simulink model "MPPT_50W_Extendido"  (R2024b)
settings: Solver=FixedStepDiscrete  StartTime=0.0  StopTime=4  FixedStep=TsPower  RelTol=1e-3
model workspace (MAT data in the model file):
  AverageN = 500
  ConfigControl = [0 0 0.032 0 0.4 0 0.7 0.02 10 1 7 1 ... (15 elements, 1x15)]
  ControllerCfg = [0 1 0.002 1 0.5 0.02 0.85 0.02 10]
  DeltaD = 0.002
  G_profile = [0 0.001 0.002 0.003 0.004 0.005 0.006 0.007 0.008 0.009 0.01 0.011 ... (16004 elements, 4001x4)]
  ImprovedMode = 2
  Panel50W : object (value not decoded)
  Pref_profile = [0 0.001 0.002 0.003 0.004 0.005 0.006 0.007 0.008 0.009 0.01 0.011 ... (8002 elements, 4001x2)]
  R_profile = [0 0.001 0.002 0.003 0.004 0.005 0.006 0.007 0.008 0.009 0.01 0.011 ... (8002 elements, 4001x2)]
  Rnorm = 6.66058394161
  T_profile = [0  25; 4  25]
  TsMPPT = 0.002
  TsPower = 2e-06
  UseAdaptiveStep = 1
  cfg_profile : timeseries (value not decoded)
libraries: spsDiodeLib x4, spsSeriesRLCBranchLib x3, spsPVArrayLib x3, spsCurrentMeasurementLib x2, spsMosfetLib x1, spsVoltageMeasurementLib x1, spsVariableResistorLib x1, spspowerguiLib x1
(part 2 of 2)

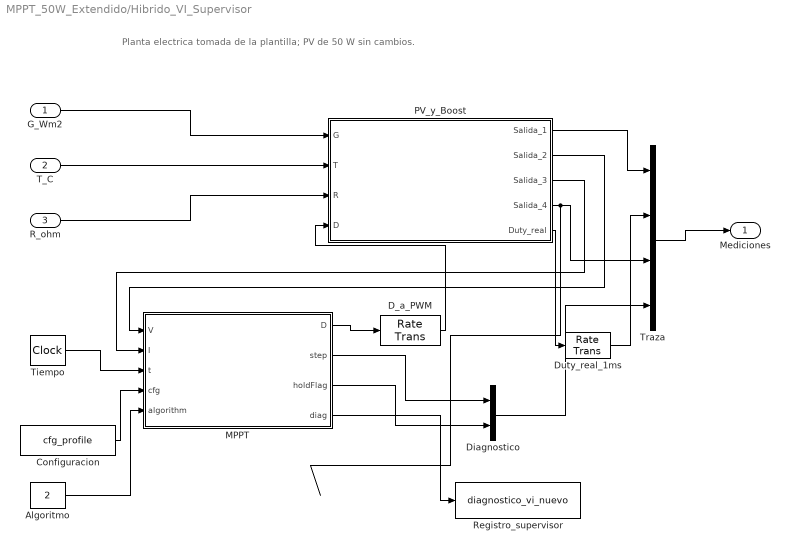
== system MPPT_50W_Extendido/Hibrido_VI_Supervisor ==
  note: Planta electrica tomada de la plantilla; PV de 50 W sin cambios.
  G_Wm2 : Inport
  T_C : Inport  Port=2
  R_ohm : Inport  Port=3
  Algoritmo : Constant  Value=2
  Configuracion : FromWorkspace  VariableName=cfg_profile  SampleTime=TsMPPT  Interpolate=off  OutputAfterFinalValue=Holding final value
  D_a_PWM : RateTransition  OutPortSampleTime=TsMPPT
  Diagnostico : Mux  Inputs=2
  Duty_real_1ms : RateTransition  OutPortSampleTime=TsMPPT
  MPPT : MATLAB Function  TreatAsAtomicUnit=on
  PV_y_Boost : Subsystem
  Registro_supervisor : ToWorkspace  VariableName=diagnostico_vi_nuevo  SaveFormat=Timeseries  SampleTime=-1
  Tiempo : DigitalClock  SampleTime=TsMPPT
  Traza : Mux
  Mediciones : Outport
  wires:
  ? -> ?
  Duty_real_1ms/1 -> Traza/2
  PV_y_Boost/5(Duty_real) -> Duty_real_1ms/1
  Traza/1 -> Mediciones/1
  Diagnostico/1 -> Traza/4
  MPPT/3(holdFlag) -> Diagnostico/2
  MPPT/2(step) -> Diagnostico/1
  PV_y_Boost/4(Salida_4) -> Traza/3
  PV_y_Boost/1(Salida_1) -> Traza/1
  D_a_PWM/1 -> PV_y_Boost/4(D)
  MPPT/1(D) -> D_a_PWM/1
  Algoritmo/1 -> MPPT/5(algorithm)
  Tiempo/1 -> MPPT/3(t)
  PV_y_Boost/3(Salida_3) -> MPPT/2(I)
  PV_y_Boost/2(Salida_2) -> MPPT/1(V)
  R_ohm/1 -> PV_y_Boost/3(R)
  T_C/1 -> PV_y_Boost/2(T)
  G_Wm2/1 -> PV_y_Boost/1(G)
  MPPT/4(diag) -> Registro_supervisor/1
  Configuracion/1 -> MPPT/4(cfg)

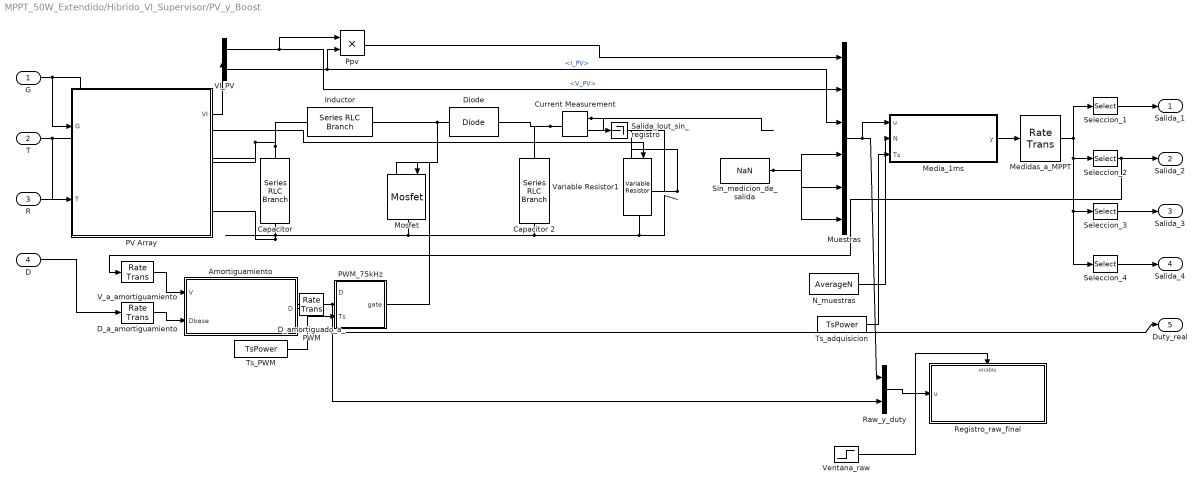
== system MPPT_50W_Extendido/Hibrido_VI_Supervisor/PV_y_Boost ==
  G : Inport
  T : Inport  Port=2
  R : Inport  Port=3
  D : Inport  Port=4
  Amortiguamiento : MATLAB Function  TreatAsAtomicUnit=on
  Capacitor : spsSeriesRLCBranchLib/Series RLC Branch  LConnTagsString=__new0  RConnTagsString=__new0  BranchType=C  Resistance=1e-4  Inductance=2e-3  SetiL0=off  InitialCurrent=5  Capacitance=2e-3  Setx0=off  InitialVoltage=0  Measurements=None
  Capacitor 2 : spsSeriesRLCBranchLib/Series RLC Branch  LConnTagsString=__new0  RConnTagsString=__new0  BranchType=C  Resistance=1e-4  Inductance=2e-3  SetiL0=off  InitialCurrent=5  Capacitance=2e-3  Setx0=off  InitialVoltage=0  Measurements=None
  Current Measurement : spsCurrentMeasurementLib/Current Measurement  PhasorSimulation=off  OutputType=Complex  PSBequivalent=0
  D_a_amortiguamiento : RateTransition  OutPortSampleTime=TsMPPT
  D_amortiguado_a_PWM : RateTransition  Deterministic=off  OutPortSampleTime=TsPower
  Diode : spsDiodeLib/Diode  Ron=0.001  Lon=0  Vf=0.1  IC=0  UseSnubber=off  Rs=500  Cs=250e-9  Measurements=off
  Inductor : spsSeriesRLCBranchLib/Series RLC Branch  LConnTagsString=__new0  RConnTagsString=__new0  BranchType=L  Resistance=0.1  Inductance=2.2e-3  SetiL0=off  InitialCurrent=5  Capacitance=1e-6  Setx0=off  InitialVoltage=0  Measurements=None
  Media_1ms : MATLAB Function  TreatAsAtomicUnit=on
  Medidas_a_MPPT : RateTransition  OutPortSampleTime=TsMPPT
  Mosfet : spsMosfetLib/Mosfet  Ron=0.01  Lon=0  Rd=0.01  Vfd=0  IC=0  Rs=1e5  Cs=inf  Measurements=off
  Muestras : Mux  Inputs=6
  N_muestras : Constant  Value=AverageN
  PV Array : Subsystem
  PWM_75kHz : MATLAB Function  TreatAsAtomicUnit=on
  Ppv : Product
  Raw_y_duty : Mux  Inputs=2
  Registro_raw_final : Subsystem
  Salida_Iout_sin_registro : Terminator
  Seleccion_1 : Selector  InputPortWidth=6  IndexOptions=Index vector (dialog)  Indices=[1 2 3]  OutputSizes=1
  Seleccion_2 : Selector  InputPortWidth=6  IndexOptions=Index vector (dialog)  Indices=2  OutputSizes=1
  Seleccion_3 : Selector  InputPortWidth=6  IndexOptions=Index vector (dialog)  Indices=3  OutputSizes=1
  Seleccion_4 : Selector  InputPortWidth=6  IndexOptions=Index vector (dialog)  Indices=[4 5 6]  OutputSizes=1
  Sin_medicion_de_salida : Constant  Value=NaN
  Ts_PWM : Constant  Value=TsPower
  Ts_adquisicion : Constant  Value=TsPower
  VI_PV : BusSelector  OutputSignals=V_PV,I_PV
  V_a_amortiguamiento : RateTransition  OutPortSampleTime=TsMPPT
  Variable Resistor1 : spsVariableResistorLib/Variable Resistor  Rabsmin=1e-3
      settings: LibrarySourceBlock=sps_lib/Passives/Variable Resistor
  Ventana_raw : Step  Time=3.8  SampleTime=2e-6
  Salida_1 : Outport
  Salida_2 : Outport  Port=2
  Salida_3 : Outport  Port=3
  Salida_4 : Outport  Port=4
  Duty_real : Outport  Port=5
  wires:
  Ts_adquisicion/1 -> Media_1ms/3(Ts)
  PWM_75kHz/1(gate) -> Mosfet/1
  Ts_PWM/1 -> PWM_75kHz/2(Ts)
  PV Array/1(VI) -> VI_PV/1
  Ventana_raw/1 -> Registro_raw_final/Enable
  Raw_y_duty/1 -> Registro_raw_final/1(u)
  D_amortiguado_a_PWM/1 -> PWM_75kHz/1(D), Raw_y_duty/2, Duty_real/1
  Amortiguamiento/1(D) -> D_amortiguado_a_PWM/1
  D_a_amortiguamiento/1 -> Amortiguamiento/2(Dbase)
  V_a_amortiguamiento/1 -> Amortiguamiento/1(V)
  D/1 -> D_a_amortiguamiento/1
  Seleccion_4/1 -> Salida_4/1
  Seleccion_3/1 -> Salida_3/1
  Seleccion_2/1 -> V_a_amortiguamiento/1, Salida_2/1
  Seleccion_1/1 -> Salida_1/1
  Medidas_a_MPPT/1 -> Seleccion_1/1, Seleccion_2/1, Seleccion_4/1, Seleccion_3/1
  Media_1ms/1(y) -> Medidas_a_MPPT/1
  N_muestras/1 -> Media_1ms/2(N)
  Muestras/1 -> Raw_y_duty/1, Media_1ms/1(u)
  Ppv/1 -> Muestras/1
  Current Measurement/1 -> Salida_Iout_sin_registro/1
  ? -> ?
  VI_PV/2 -> Muestras/3, Ppv/2  "<I_PV>"
  VI_PV/1 -> Muestras/2, Ppv/1  "<V_PV>"
  R/1 -> Variable Resistor1/1
  T/1 -> PV Array/2(T)
  G/1 -> PV Array/1(G)
  Sin_medicion_de_salida/1 -> Muestras/4, Muestras/5, Muestras/6
  connections:
  Capacitor/RConn1 -- PV Array/RConn2 -- Capacitor 2/RConn1 -- Variable Resistor1/RConn1 -- Mosfet/RConn1
  Current Measurement/RConn1 -- Variable Resistor1/LConn1
  Current Measurement/LConn1 -- Diode/RConn1 -- Capacitor 2/LConn1
  Diode/LConn1 -- Inductor/RConn1 -- Mosfet/LConn1
  Capacitor/LConn1 -- PV Array/RConn1 -- Inductor/LConn1

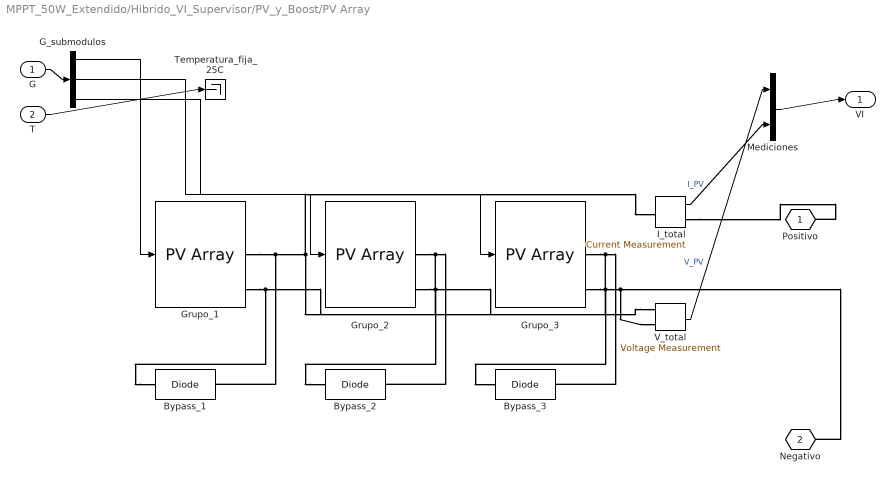
== system MPPT_50W_Extendido/Hibrido_VI_Supervisor/PV_y_Boost/PV Array ==
  G : Inport
  T : Inport  Port=2
  Bypass_1 : spsDiodeLib/Diode  Ron=.001  Lon=0  Vf=.3  IC=0  UseSnubber=off  Rs=500  Cs=250e-9  Measurements=off
  Bypass_2 : spsDiodeLib/Diode  Ron=.001  Lon=0  Vf=.3  IC=0  UseSnubber=off  Rs=500  Cs=250e-9  Measurements=off
  Bypass_3 : spsDiodeLib/Diode  Ron=.001  Lon=0  Vf=.3  IC=0  UseSnubber=off  Rs=500  Cs=250e-9  Measurements=off
  G_submodulos : Demux  Outputs=3
  Grupo_1 : spsPVArrayLib/PV Array  Npar=1  Nser=1  PlotType=array @ 25 deg.C & specified irradiances  S_vec="[ 1000  500  100 ]"  Temp_C_vec=[1000 900 800]  ModuleName=User-defined  PlotWhenSelected=off  Pm=16.6683  Ncell=11  Voc=7.52  Isc=2.79  Vm=6.083333333333333  Im=2.74  beta_Voc_pc=-0.30  alpha_Isc_pc=0.046  beta_Voc=-0.02256  alpha_Isc=0.0012834  IL=2.8521  I0=9.4809e-12  nI=1.0068  Rsh=6554.1264  Rs=0.21261  RobustModel=on  RobustCellTemperature=25  BAL=on  Tc=1e-6  Tfilter=5e-5
  Grupo_2 : spsPVArrayLib/PV Array  Npar=1  Nser=1  PlotType=array @ 25 deg.C & specified irradiances  S_vec="[ 1000  500  100 ]"  Temp_C_vec=[1000 900 800]  ModuleName=User-defined  PlotWhenSelected=off  Pm=16.6683  Ncell=11  Voc=7.52  Isc=2.79  Vm=6.083333333333333  Im=2.74  beta_Voc_pc=-0.30  alpha_Isc_pc=0.046  beta_Voc=-0.02256  alpha_Isc=0.0012834  IL=2.8521  I0=9.4809e-12  nI=1.0068  Rsh=6554.1264  Rs=0.21261  RobustModel=on  RobustCellTemperature=25  BAL=on  Tc=1e-6  Tfilter=5e-5
  Grupo_3 : spsPVArrayLib/PV Array  Npar=1  Nser=1  PlotType=array @ 25 deg.C & specified irradiances  S_vec="[ 1000  500  100 ]"  Temp_C_vec=[1000 900 800]  ModuleName=User-defined  PlotWhenSelected=off  Pm=16.6683  Ncell=11  Voc=7.52  Isc=2.79  Vm=6.083333333333333  Im=2.74  beta_Voc_pc=-0.30  alpha_Isc_pc=0.046  beta_Voc=-0.02256  alpha_Isc=0.0012834  IL=2.8521  I0=9.4809e-12  nI=1.0068  Rsh=6554.1264  Rs=0.21261  RobustModel=on  RobustCellTemperature=25  BAL=on  Tc=1e-6  Tfilter=5e-5
  I_total : spsCurrentMeasurementLib/Current Measurement  PhasorSimulation=off  OutputType=Complex  PSBequivalent=0
  Mediciones : BusCreator  Inputs=2
  Temperatura_fija_25C : Terminator
  V_total : spsVoltageMeasurementLib/Voltage Measurement  PhasorSimulation=off  OutputType=Complex  PSBequivalent=0
  Positivo : PMIOPort  Side=Right
  Negativo : PMIOPort  Port=2  Side=Right
  VI : Outport
  wires:
  Mediciones/1 -> VI/1
  I_total/1 -> Mediciones/2  "I_PV"
  V_total/1 -> Mediciones/1  "V_PV"
  G_submodulos/3 -> Grupo_3/1
  G_submodulos/2 -> Grupo_2/1
  G_submodulos/1 -> Grupo_1/1
  T/1 -> Temperatura_fija_25C/1
  G/1 -> G_submodulos/1
  connections:
  I_total/RConn1 -- Positivo/RConn1
  Bypass_2/LConn1 -- Grupo_2/RConn2 -- Grupo_3/RConn1 -- Bypass_3/RConn1
  V_total/LConn2 -- Negativo/RConn1 -- Grupo_3/RConn2 -- Bypass_3/LConn1
  Bypass_1/LConn1 -- Grupo_1/RConn2 -- Grupo_2/RConn1 -- Bypass_2/RConn1
  V_total/LConn1 -- I_total/LConn1 -- Grupo_1/RConn1 -- Bypass_1/RConn1

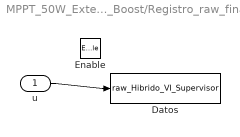
== system MPPT_50W_Extendido/Hibrido_VI_Supervisor/PV_y_Boost/Registro_raw_final ==
  u : Inport
  Enable : EnablePort
  Datos : ToWorkspace  VariableName=raw_Hibrido_VI_Supervisor  SaveFormat=Timeseries  SampleTime=2e-6
  wires:
  u/1 -> Datos/1

== matlab function MPPT_50W_Extendido/Hibrido_VI_Supervisor/MPPT ==
  settings: updateMethod=DISCRETE  sampleTime=TsMPPT
  data: V input; D output; I input; t input; cfg input; algorithm input; step output; holdFlag output; diag output
function [D,step,holdFlag,diag]=mppt_extendido_50w(V,I,t,cfg,algorithm)
%#codegen
% MPPT at 2 ms. V and I are the only measurements. t is a local clock.
% Diagnostic phases: 0 wait, 1 scan, 2 recover, 3 hold, 4 refine.
% cfg(9)=0 is reserved for an ablation without global search.
% cfg(10) is the scout interval in seconds. Zero disables only scouts.
% diag(5) gives the exploration type: 1 full, 2 short scout, 3 deep scout.
persistent priorLocalDP pausedLast resumeDirection failedScoutCount
persistent phase entered d vRef beforeEventV pendingAudit lastAudit
persistent lastScout kind shortNext lowerVoltageNext
persistent previousV previousP vFilt pFast iFast pSlow iSlow eventCount
persistent localStarted direction ringV ringP ringD ringNext ringCount
persistent incumbentV incumbentP incumbentD firstEdge secondEdge leg edgeCount
persistent bestScore bestV bestD measuredD targetD testPeak approach confirmCount confirmPower

% cfg(11): 0 PO, 1 INC, 2 Meng literal, 3 original scout, 4 integrated.
% cfg(12): two-step gate; cfg(13): adaptive V/I step.
% cfg(14): integration step cap (literal Meng always uses 0.05).
% mode 5: pilot with a 0.00035 floor; mode 6 retains the paper floor 0.002.
% Both are normalized by nameplate resistance cfg(15); pauses last one tick.
if cfg(11)==7
    [D,step,holdFlag,diag]=fastLocal(V,I,t,cfg);
    return
end
if cfg(11)<3
    [D,step,holdFlag,diag]=localArticle(V,I,t,cfg);
    return
end
lower=cfg(6);
upper=floor(1024*cfg(7))/1024;
if isempty(phase)
    priorLocalDP=0;pausedLast=false;resumeDirection=-1;failedScoutCount=0;phase=0;entered=t;d=cfg(5);vRef=0;beforeEventV=0;
    pendingAudit=false;lastAudit=0;
    lastScout=0;kind=0;shortNext=true;lowerVoltageNext=true;
    previousV=V;previousP=V*I;vFilt=V;
    pFast=V*I;iFast=I;pSlow=pFast;iSlow=I;eventCount=0;
    localStarted=false;direction=-1;
    ringV=zeros(32,1);ringP=zeros(32,1);ringD=zeros(32,1);
    ringNext=1;ringCount=0;
    incumbentV=0;incumbentP=0;incumbentD=d;
    firstEdge=0;secondEdge=0;leg=1;edgeCount=0;
    bestScore=0;bestV=0;bestD=d;measuredD=d;targetD=d;
    testPeak=false;approach=false;confirmCount=0;confirmPower=0;
end
P=V*I;
D=d;step=0;holdFlag=double(phase==3);
lowRegion=vRef>0 && vRef<=8.5;
eligibleRegion=vRef>0 && (vRef<15 || d>=.58);
diag=[min(phase,4) double(phase==1) vRef 0 kind double(eligibleRegion)];
if phase==5,diag(1)=2;end
if algorithm<0 || ~isfinite(P) || V<.10 || I<.001,return;end

oldD=d;
oldVFilt=vFilt;
vFilt=vFilt+.30*(V-vFilt);
pFast=pFast+.20*(P-pFast);
iFast=iFast+.20*(I-iFast);
trigger=0;
if phase==0 && t>=cfg(8)
    phase=4;entered=t;
end

if phase==4
    % Local hill climb during acquisition and after confirmed disturbance.
    % A 64 ms window screens drift before committing to a voltage reference.
    ringV(ringNext)=V;ringP(ringNext)=P;ringD(ringNext)=d;
    ringNext=mod(ringNext,32)+1;
    ringCount=min(32,ringCount+1);
    deltaP=P-previousP;
    newLocal=~localStarted;
    if cfg(11)>=8
        if newLocal
            localStarted=true;priorLocalDP=0;pausedLast=false;resumeDirection=-1;
        end
        [direction,localStep,pausedLast,resumeDirection]=fastRule( ...
            V,I,previousV,previousP,priorLocalDP,pausedLast,resumeDirection,newLocal,cfg);
    else
    deltaP=P-previousP;
    newLocal=~localStarted;
    if ~localStarted
        direction=-1;
        localStarted=true;
        priorLocalDP=0;pausedLast=false;resumeDirection=-1;
    elseif deltaP~=0
        if (P>previousP)==(V>previousV),direction=-1;else,direction=1;end
        % Literal Algorithm 2: all four branches require prior deltaP>0.
        if cfg(11)==4 && cfg(12)>0 && priorLocalDP<=0,direction=0;end
    else
        direction=0;
    end
    % Integration guard: the literal two-step pause lasts at most one tick.
    % A fresh physical perturbation is then required; a flat quantized sample
    % alone is not evidence that a maximum has been found.
    if cfg(11)>=5 && ~newLocal && cfg(12)>0
        if pausedLast
            if direction==0,direction=resumeDirection;end
            pausedLast=false;
        elseif priorLocalDP<=0
            if direction~=0,resumeDirection=direction;end
            direction=0;pausedLast=true;
        end
    end
    if direction~=0,resumeDirection=direction;end
    localStep=cfg(3);
    if cfg(11)==4 && cfg(13)>0
        localStep=clamp((V/max(I,.001))*cfg(3),.002,cfg(14));
    elseif cfg(11)>=5 && cfg(13)>0
        minimum=.00035;if cfg(11)==6,minimum=.002;end
        localStep=clamp((V/max(I,.001))/cfg(15)*cfg(3),minimum,cfg(14));
    end
    end
    priorLocalDP=deltaP;
    d=clamp(d+direction*localStep,lower,upper);
    minimumRefine=.12;if cfg(11)>=8,minimumRefine=.08;end
    if ringCount==32 && t-entered>=minimumRefine
        [quiet,centerV,centerP,centerD]=quietWindow(ringV,ringP,ringD,ringNext);
        if quiet
            pendingAudit=beforeEventV>0 && ...
                abs(centerV-beforeEventV)>max(1.0,.18*beforeEventV);
            beforeEventV=0;
            vRef=centerV;d=centerD;pSlow=centerP;iSlow=centerP/centerV;
            pFast=P;iFast=I;eventCount=0;
            phase=3;entered=t;kind=0;
        end
    end
elseif phase==3
    % Voltage servo and a fast/slow detector. Gradual drift updates its anchors.
    % A queued event is relevant only near the quiet point that armed it.
    if t-entered>.250,pendingAudit=false;end
    e=vFilt-vRef;
    if cfg(11)>=8
        d=voltageStep(d,e,vRef,.0030,.0060,lower,upper);
    else
        d=voltageStep(d,e,vRef,.0016,.0035,lower,upper);
    end
    relativeP=abs(pFast-pSlow)/max(.5,.105*pSlow);
    relativeI=abs(iFast-iSlow)/max(.045,.13*iSlow);
    deviation=max(abs(e)/.80,min(relativeP,relativeI));
    if deviation>=1 && t-entered>=.050
        eventCount=eventCount+1;
    elseif deviation<.65
        eventCount=0;
    else
        eventCount=max(0,eventCount-1);
    end
    if eventCount<2
        pSlow=pSlow+.035*(P-pSlow);
        iSlow=iSlow+.035*(I-iSlow);
    end
    if eventCount>=4
        if cfg(11)>=8,failedScoutCount=0;end
        beforeEventV=vRef;
        eventCount=0;entered=t;
        ringCount=0;ringNext=1;localStarted=false;
        % Opposing V/I movement is consistent with restoring this reference.
        % This test does not identify the physical cause of the disturbance.
        if abs(e)>.65 && abs(iFast-iSlow)>.020 && e*(iFast-iSlow)<0
            phase=5;
        else
            phase=4;
        end
    elseif cfg(9)>0 && t-entered>=.050 && deviation<.65
        voltageReady=abs(e)<max(.18,.02*vRef);
        % The voltage target may be unreachable at the upper PWM limit.
        % Stable measured P/I permit probing toward lower duty from that limit.
        clampedReady=oldD>=upper-.002 && e>0 && ...
            abs(iFast-iSlow)<max(.015,.03*iSlow);
        auditInterval=4.0;effectiveScout=cfg(10);
        if cfg(11)>=8
            auditInterval=6.0;
            effectiveScout=cfg(10)*min(3,1+floor(failedScoutCount/2));
        end
        fullDue=voltageReady && ...
            (t-lastAudit>=auditInterval || (pendingAudit && t-lastAudit>=1.20));
        scoutDue=cfg(10)>0 && eligibleRegion && ~pendingAudit && t-lastScout>=effectiveScout && ...
            (voltageReady || clampedReady) && abs(pFast-pSlow)<max(.12,.03*pSlow) && ...
            (~lowRegion || oldD-lower>=.06);
        if fullDue || scoutDue
            phase=1;entered=t;lastScout=t;trigger=1;
            pendingAudit=false;
            incumbentV=vRef;incumbentP=pSlow;incumbentD=oldD;
            leg=1;edgeCount=0;bestScore=0;bestV=0;bestD=d;
            if fullDue
                kind=1;lastAudit=t;
                if d-lower<=upper-d
                    firstEdge=lower;secondEdge=upper;
                else
                    firstEdge=upper;secondEdge=lower;
                end
            elseif lowRegion
                kind=3;
                if shortNext,kind=2;end
                shortNext=~shortNext;
                firstEdge=lower;
            else
                kind=3;
                if (lowerVoltageNext && upper-d>=.06) || d-lower<.06
                    firstEdge=upper;
                else
                    firstEdge=lower;
                end
                lowerVoltageNext=~lowerVoltageNext;
            end
        end
    end
elseif phase==5
    % Brief, bounded recovery around the last reference with voltage lead.
    e=vFilt-vRef;
    lead=e+3*(vFilt-oldVFilt);
    d=voltageStep(d,lead,vRef,.0030,.0060,lower,upper);
    if (t-entered>=.018 && abs(e)<.30) || t-entered>=.082
        phase=4;entered=t;
    end
elseif phase==1
    % A full audit covers both ends. A scout visits just one voltage side.
    separated=abs(V-incumbentV)>=max(.45,.12*incumbentV);
    nearby=abs(V-previousV)<=max(.30,.065*V);
    score=min(P,previousP);
    if t-entered>=.010 && separated && nearby && score>bestScore
        bestScore=score;bestV=.5*(V+previousV);bestD=.5*(d+measuredD);
    end
    edge=firstEdge;
    if leg==2,edge=secondEdge;end
    scanSlew=.018;if cfg(11)>=8,scanSlew=.030;end
    d=d+clamp(edge-d,-scanSlew,scanSlew);
    if abs(d-edge)<1e-9,edgeCount=edgeCount+1;else,edgeCount=0;end
    % A shallow scout samples beyond the local lobe, then returns if no
    % advantage is visible. Its paired deep scout covers the rest of that side.
    shallowDecline=V-incumbentV>=.50 && score<.80*incumbentP;
    shallowExtent=V-incumbentV>=max(2.4,.35*incumbentV);
    shallowDone=kind==2 && (shallowDecline || shallowExtent) && ...
        bestScore<=incumbentP+margin(incumbentP);
    if edgeCount>=7 || shallowDone
        if kind==1 && leg==1
            leg=2;edgeCount=0;
        else
            phase=2;entered=t;
            testPeak=bestScore>incumbentP+margin(incumbentP);
            if testPeak
                vRef=bestV;targetD=bestD;
            else
                vRef=incumbentV;targetD=incumbentD;
            end
            approach=true;confirmCount=0;confirmPower=0;
        end
    end
elseif phase==2
    % Revisit the measured candidate. A settled confirmation prevents
    % accepting a transient as an improved equilibrium point.
    if approach
        returnSlew=.018;if cfg(11)>=8,returnSlew=.030;end
        d=d+clamp(targetD-d,-returnSlew,returnSlew);
        approach=abs(d-targetD)>.001;
    else
        e=vFilt-vRef;
        lead=e+3*(vFilt-oldVFilt);
        if cfg(11)>=8
            d=voltageStep(d,lead,vRef,.0040,.0100,lower,upper);
        else
            d=voltageStep(d,lead,vRef,.0025,.0060,lower,upper);
        end
        if abs(e)<max(.18,.018*vRef) && abs(vFilt-oldVFilt)<.07
            confirmCount=confirmCount+1;confirmPower=confirmPower+P;
        else
            confirmCount=0;confirmPower=0;
        end
    end
    confirmed=confirmCount>=8;
    expired=t-entered>=.260;
    if confirmed || expired
        if cfg(11)>=8 && kind>=2
            if testPeak && confirmed && confirmPower/max(1,confirmCount)>incumbentP+margin(incumbentP)
                failedScoutCount=0;
            elseif ~testPeak && confirmed
                failedScoutCount=min(6,failedScoutCount+1);
            end
        end
        if testPeak && (~confirmed || confirmPower/max(1,confirmCount)<=incumbentP+margin(incumbentP))
            vRef=incumbentV;targetD=incumbentD;
            testPeak=false;approach=true;entered=t;
            confirmCount=0;confirmPower=0;
        elseif confirmed && ~testPeak && abs(confirmPower/confirmCount-incumbentP)<=margin(incumbentP)
            phase=3;entered=t;kind=0;pSlow=confirmPower/confirmCount;iSlow=I;
            pFast=P;iFast=I;eventCount=0;
        else
            phase=4;entered=t;
            ringCount=0;ringNext=1;localStarted=false;beforeEventV=0;
        end
    end
end

measuredD=oldD;previousV=V;previousP=P;
D=clamp(d,lower,upper);d=D;step=D-oldD;
holdFlag=double(phase==3);
reportedPhase=phase;
if phase==5,reportedPhase=2;end
diag=[reportedPhase double(phase==1) vRef trigger kind double(eligibleRegion)];
end

function [quiet,V,P,D]=quietWindow(v,p,d,next)
sumOldV=0;sumOldP=0;sumV=0;sumP=0;sumD=0;
for k=0:15
    earlier=mod(next-1+k,32)+1;
    later=mod(next+15+k,32)+1;
    sumOldV=sumOldV+v(earlier);sumOldP=sumOldP+p(earlier);
    sumV=sumV+v(later);sumP=sumP+p(later);sumD=sumD+d(later);
end
V=sumV/16;P=sumP/16;D=sumD/16;
quiet=abs(P-sumOldP/16)<=max(.09,.011*P) && ...
    abs(V-sumOldV/16)<=max(.07,.011*V) && ...
    max(d)-min(d)<=.016 && max(v)-min(v)<=.80;
end

function next=voltageStep(d,error,reference,gain,slew,lo,hi)
if abs(error)>max(.035,.0025*reference)
    next=clamp(d+clamp(gain*error,-slew,slew),lo,hi);
else
    next=d;
end
end

function required=margin(P)
required=max(.08,.012*P);
end

function bounded=clamp(x,lo,hi)
bounded=min(hi,max(lo,x));
end

function [D,step,holdFlag,diag]=localArticle(V,I,t,cfg)
% Direct transcription of Algorithm 2 (p.5332), with section 3.3 step.
% Startup seed and singularity guard are implementation conventions.
persistent d v1 p1 p2 started
if isempty(d),d=cfg(5);v1=V;p1=V*I;p2=p1;started=false;end
P=V*I; dp=P-p1; dpPrevious=p1-p2; dv=V-v1;
old=d; direction=0; h=cfg(3);
lo=cfg(6);hi=floor(1024*cfg(7))/1024;
if t>=cfg(8) && isfinite(P) && V>=.10 && I>=.001
    if ~started
        direction=-1; started=true;
    elseif cfg(11)==1
        if abs(dv)>1e-4
            slope=I+V*(I-p1/max(v1,.1))/dv;
            if slope>.002,direction=-1;elseif slope<-.002,direction=1;end
        else
            di=I-p1/max(v1,.1);
            if di>1e-5,direction=-1;elseif di<-1e-5,direction=1;end
        end
    elseif dp~=0
        if (dp>0)==(dv>0),direction=-1;else,direction=1;end
        if cfg(11)==2 && cfg(12)>0 && dpPrevious<=0,direction=0;end
    end
    if cfg(11)==2 && cfg(13)>0,h=clamp(V/max(I,.001)*cfg(3),.002,.05);end
    d=clamp(d+direction*h,lo,hi);
end
p2=p1;p1=P;v1=V;
D=d;step=d-old;holdFlag=double(started && direction==0);
diag=[4 0 0 0 0 0];
end


function [D,step,holdFlag,diag]=fastLocal(V,I,t,cfg)
% Own extension of the two-increment/V-I rule; not the Meng replica.
persistent d previousV previousP previousDP paused resume started
if isempty(d)
    d=cfg(5);previousV=V;previousP=V*I;previousDP=0;
    paused=false;resume=-1;started=false;
end
old=d;P=V*I;direction=0;
if t>=cfg(8) && isfinite(P) && V>=.10 && I>=.001
    [direction,h,paused,resume]=fastRule(V,I,previousV,previousP,previousDP,paused,resume,~started,cfg);
    started=true;
    d=clamp(d+direction*h,cfg(6),floor(1024*cfg(7))/1024);
end
previousDP=P-previousP;previousP=P;previousV=V;
D=d;step=d-old;holdFlag=double(started && direction==0);diag=[4 0 0 0 0 0];
end

function [direction,h,paused,resume]=fastRule(V,I,oldV,oldP,priorDP,paused,resume,newLocal,cfg)
% V/I normalization, measured normalized slope and a bounded trust factor.
% All decisions use current/past V and I plus fixed nameplate constants.
persistent trust lastDirection
if isempty(trust) || newLocal,trust=1;lastDirection=-1;end
P=V*I;dp=P-oldP;dv=V-oldV;
if newLocal
    direction=-1;relativeSlope=1;paused=false;resume=-1;
else
    if abs(dv)>.0025
        slope=dp/dv;
        direction=-sign(slope);
        relativeSlope=min(1.5,abs(slope)/max(I,.05));
    else
        direction=resume;relativeSlope=.025;
    end
    if direction==0,direction=resume;end
    if abs(dp)>max(.5,.12*P),trust=max(trust,.5);end
    if direction~=lastDirection
        trust=max(.03,.55*trust);
    else
        trust=min(1,1.12*trust);
    end
end
resistanceScale=sqrt(clamp((V/max(I,.001))/cfg(15),.25,4));
h=clamp(cfg(3)*resistanceScale*max(.015,relativeSlope)*trust,.00015,.040);
if cfg(13)<=0,h=.004;end
if ~newLocal && cfg(12)>0 && relativeSlope<.50
    if paused
        paused=false;
    elseif dp*priorDP<=0
        resume=direction;direction=0;paused=true;
    end
else
    paused=false;
end
if direction~=0,resume=direction;lastDirection=direction;end
end

== matlab function MPPT_50W_Extendido/Hibrido_VI_Supervisor/PV_y_Boost/Amortiguamiento ==
  settings: updateMethod=DISCRETE  sampleTime=TsMPPT
  data: V input; D output; Dbase input
function D=amortiguamiento_vi_muestreado(V,Dbase)
%#codegen
% Only the same sampled INA226 input voltage reaches this block.
persistent Vf
if isempty(Vf),Vf=V;end
Ts=.002;a=exp(-Ts/.002);
Vf=a*Vf+(1-a)*V;
trim=min(.04,max(-.04,0.0040000000000000001*(V-Vf)));
D=min(.70,max(0,Dbase+trim));
end

== matlab function MPPT_50W_Extendido/Hibrido_VI_Supervisor/PV_y_Boost/Media_1ms ==
  settings: updateMethod=DISCRETE  sampleTime=TsPower
  data: u input; y output; N input; Ts input
function y=medicion_ina_vi(u,N,Ts)
%#codegen
% Evaluation P/Vo retain independent 1 ms block means.
% Controller V/I emulate triggered INA226: shunt then bus, AVG=1/140 us.
% Software readout budget assumed 1 ms; start a new pair every 2 ms.
% Quantization uses the provided 0.01 ohm shunt. No random noise assumed.
persistent s n last tick sumI sumV heldI heldV delivered
if isempty(tick)
    s=zeros(6,1);n=0;last=zeros(6,1);tick=0;
    sumI=0;sumV=0;heldI=0;heldV=0;delivered=false;
end
s=s+u;n=n+1;
if n>=N,last=s/n;n=0;s=zeros(6,1);end
period=max(1,round(.002/Ts));ct=max(1,round(.000140/Ts));
ready=max(2*ct,round(.001/Ts));k=mod(tick,period);
if k==0,sumI=0;sumV=0;delivered=false;end
if k<ct
    sumI=sumI+u(3);
elseif k<2*ct
    sumV=sumV+u(2);
end
if k>=ready && ~delivered
    heldI=.00025*round((sumI/ct)/.00025);
    heldV=.00125*round((sumV/ct)/.00125);
    delivered=true;
end
last(2)=heldV;last(3)=heldI;y=last;tick=tick+1;
end

== matlab function MPPT_50W_Extendido/Hibrido_VI_Supervisor/PV_y_Boost/PWM_75kHz ==
  settings: updateMethod=DISCRETE  sampleTime=TsPower
  data: D input; gate output; Ts input
function gate=pwm_fraccional_12k(D,Ts)
%#codegen
% Fractional-period DPWM with accumulated on-time error, common to all branches.
% Average switching frequency = 12 kHz; duty error does not accumulate.
persistent remaining onLeft periodError dutyError
if isempty(remaining)
    remaining=0;onLeft=0;periodError=0;dutyError=0;
end
D=min(floor(.70*1024),max(0,round(1024*D)))/1024;
if remaining<=0
    target=1/(75000*Ts)+periodError;
    ticks=max(2,floor(target));periodError=target-ticks;
    targetOn=D*ticks+dutyError;
    onLeft=floor(targetOn);dutyError=targetOn-onLeft;
    remaining=ticks;
end
gate=double(onLeft>0);
remaining=remaining-1;onLeft=max(0,onLeft-1);
end
